simulink model "photon_dynamics"  (R2026a)
settings: Solver=FixedStepAuto  StopTime=40  FixedStep=1e-3
settings Model: Creator=celebi  LastModifiedBy=celebi

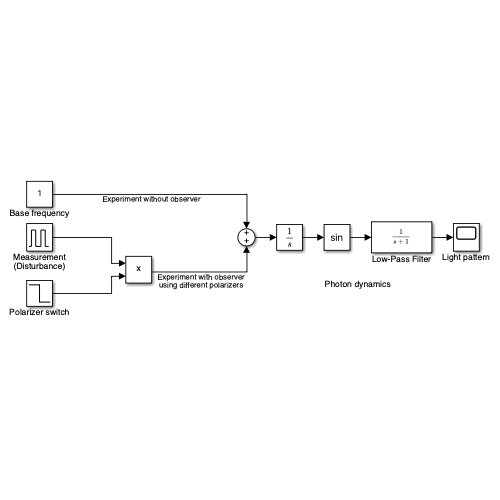
[thumbnail: Simulink's stored preview of the top-level diagram]
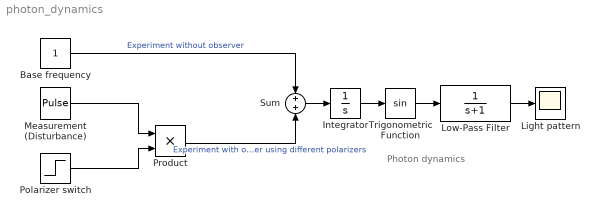
== system photon_dynamics ==
  note: Photon dynamics
  Base frequency : Constant
  Integrator : Integrator
  Light pattern : Scope
      settings: ActiveDisplayYMinimum=-0.91678592497105471  ActiveDisplayYMaximum=0.94209042387296948
  Low-Pass Filter : TransferFcn  Denominator=[1 1]
  Measurement (Disturbance) : DiscretePulseGenerator  PulseType=Time based  Amplitude=99  Period=40  PulseWidth=50  PhaseDelay=20
  Polarizer switch : Step  Time=30  InitialValue=1  FinalValue=0  SampleTime=0
  Product : Product
  Sum : Sum
  Trigonometric Function : Trigonometry
  wires:
  Base frequency/1 -> Sum/1  "Experiment without observer"
  Measurement (Disturbance)/1 -> Product/1
  Product/1 -> Sum/2  "Experiment with observer using different polarizers"
  Polarizer switch/1 -> Product/2
  Trigonometric Function/1 -> Low-Pass Filter/1
  Integrator/1 -> Trigonometric Function/1
  Low-Pass Filter/1 -> Light pattern/1
  Sum/1 -> Integrator/1
